simulink model "ids_android_app"  (R2024a)
settings: Solver=FixedStepDiscrete  StartTime=0.0  StopTime=inf  FixedStep=0.1  RelTol=1e-3
libraries: androiduilib x9, androidsensorlib x4, androidcommunicationlib x2, androidaudiovideolib x1
settings Model: Creator=prana  LastModifiedBy=prana
settings OptimizationCC: EnhancedBackFolding=on  PassReuseOutputArgsAs=Individual arguments  ZeroExternalMemoryAtStartup=off  ZeroInternalMemoryAtStartup=off  MaxStackSize=64  OptimizeBlockOrder=speed  DifferentSizesBufferReuse=on  OptimizationCustomize=off  EfficientTunableParamExpr=on
settings DebuggingCC: ParameterTunabilityLossMsg=error
settings HardwareCC: ProdBitPerPointer=32  ProdBitPerSizeT=32  ProdBitPerPtrDiffT=32  ProdLargestAtomicInteger=Long  ProdLargestAtomicFloat=Double  ProdWordSize=32  ProdHWDeviceType=ARM Compatible->ARM Cortex  UseEmbeddedCoderFeatures=off  UseSimulinkCoderFeatures=off
settings SFSimCC: MATLABDynamicMemAlloc=off
settings RTWCC: Description=Embedded Coder  SystemTargetFile=ert.tlc  HardwareBoard=Android Device  TLCOptions="-aInlineSetEventsForThisBaseRateFcn=TLC_FALSE -aSuppressMultiTaskScheduler=TLC_FALSE  -aRateBasedStepFcn=0"  TemplateMakefile=ert_default_tmf  RTWVerbose=off  Toolchain=Android SDK/NDK Tools
settings CodeAppCC: ForceParamTrailComments=on  IgnoreCustomStorageClasses=off  OperatorAnnotations=on  SimulinkDataObjDesc=on  SFDataObjDesc=on  InsertBlockDesc=on
settings ERTTargetCC: SupportNonInlinedSFcns=on

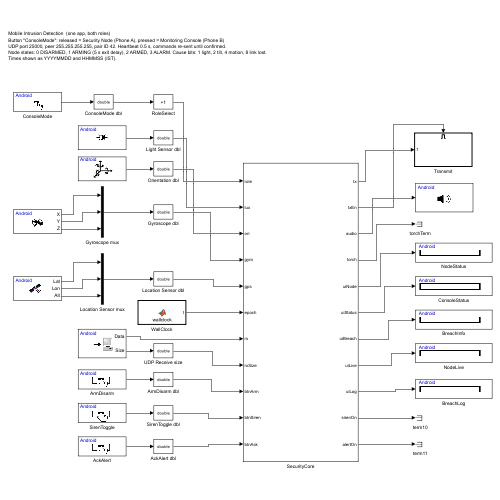
[thumbnail: Simulink's stored preview of the top-level diagram]
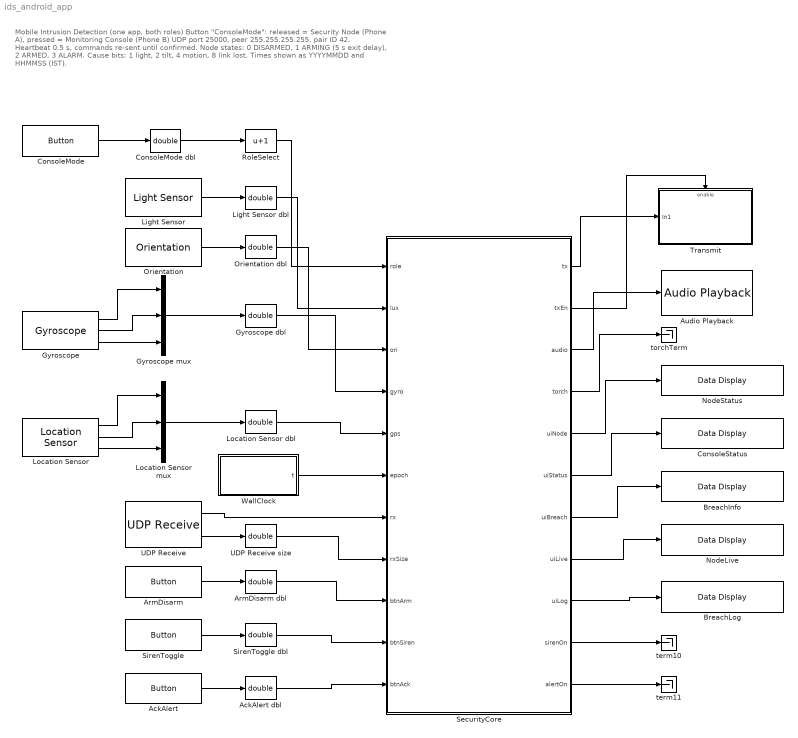
== system ids_android_app ==
  note: Mobile Intrusion Detection  (one app, both roles)
      | Button "ConsoleMode": released = Security Node (Phone A), pressed = Monitoring Console (Phone B)
      | UDP port 25000, peer 255.255.255.255, pair ID 42. Heartbeat 0.5 s, commands re-sent until confirmed.
      | Node states: 0 DISARMED, 1 ARMING (5 s exit delay), 2 ARMED, 3 ALARM. Cause bits: 1 light, 2 tilt, 4 motion, 8 link lost.
      | Times shown as YYYYMMDD and HHMMSS (IST).
  AckAlert : androiduilib/Button  ButtonState=Not pressed  ButtonId=ids_android_app/AckAlert  State=off  SampleTime=0.1  BlockPlatform=Android
  AckAlert dbl : DataTypeConversion  OutDataTypeStr=double  SaturateOnIntegerOverflow=off  RndMeth=Floor
  ArmDisarm : androiduilib/Button  ButtonState=Not pressed  ButtonId=ids_android_app/ArmDisarm  State=off  SampleTime=0.1  BlockPlatform=Android
  ArmDisarm dbl : DataTypeConversion  OutDataTypeStr=double  SaturateOnIntegerOverflow=off  RndMeth=Floor
  Audio Playback : androidaudiovideolib/Audio Playback  SampleFreq=44100  AudioSamplingFreq=44100  SampleTime=0.1  DeviceStr=0  QueueDuration=0  BlockPlatform=Android
  BreachInfo : androiduilib/Data Display  DataDisplayId=ids_android_app/BreachInfo  Format=Float  Precision=6  SimulateUsing=Code generation  blockPlatform=Android
  BreachLog : androiduilib/Data Display  DataDisplayId=ids_android_app/BreachLog  Format=Float  Precision=6  SimulateUsing=Code generation  blockPlatform=Android
  ConsoleMode : androiduilib/Button  ButtonState=Not pressed  ButtonId=ids_android_app/ConsoleMode  State=off  SampleTime=0.1  BlockPlatform=Android
  ConsoleMode dbl : DataTypeConversion  OutDataTypeStr=double  SaturateOnIntegerOverflow=off  RndMeth=Floor
  ConsoleStatus : androiduilib/Data Display  DataDisplayId=ids_android_app/ConsoleStatus  Format=Float  Precision=6  SimulateUsing=Code generation  blockPlatform=Android
  Gyroscope : androidsensorlib/Gyroscope  OutputVector=off  SampleTime=0.1  BlockPlatform=Android
  Gyroscope dbl : DataTypeConversion  OutDataTypeStr=double  SaturateOnIntegerOverflow=off  RndMeth=Floor
  Gyroscope mux : Mux  Inputs=3
  Light Sensor : androidsensorlib/Light Sensor  SampleTime=0.1  BlockPlatform=Android
  Light Sensor dbl : DataTypeConversion  OutDataTypeStr=double  SaturateOnIntegerOverflow=off  RndMeth=Floor
  Location Sensor : androidsensorlib/Location Sensor  OutputVector=off  SampleTime=0.1  BlockPlatform=Android
  Location Sensor dbl : DataTypeConversion  OutDataTypeStr=double  SaturateOnIntegerOverflow=off  RndMeth=Floor
  Location Sensor mux : Mux  Inputs=3
  NodeLive : androiduilib/Data Display  DataDisplayId=ids_android_app/NodeLive  Format=Float  Precision=6  SimulateUsing=Code generation  blockPlatform=Android
  NodeStatus : androiduilib/Data Display  DataDisplayId=ids_android_app/NodeStatus  Format=Float  Precision=6  SimulateUsing=Code generation  blockPlatform=Android
  Orientation : androidsensorlib/Orientation  SampleTime=0.1
  Orientation dbl : DataTypeConversion  OutDataTypeStr=double  SaturateOnIntegerOverflow=off  RndMeth=Floor
  RoleSelect : Bias  Bias=1  SaturateOnIntegerOverflow=off
  SecurityCore : Subsystem
  SirenToggle : androiduilib/Button  ButtonState=Not pressed  ButtonId=ids_android_app/SirenToggle  State=off  SampleTime=0.1  BlockPlatform=Android
  SirenToggle dbl : DataTypeConversion  OutDataTypeStr=double  SaturateOnIntegerOverflow=off  RndMeth=Floor
  Transmit : Subsystem  TreatAsAtomicUnit=on
  UDP Receive : androidcommunicationlib/UDP Receive  localURL='0.0.0.0'  localPort=25000  remoteURL='0.0.0.0'  remotePort=-1  recvBufferSize=1024  signalDatatype=double  dims=16  isVarSize=off  showBlockingTime=off  blockingTime=0  sampletime=0.1  blockPlatform=Android
  UDP Receive size : DataTypeConversion  OutDataTypeStr=double  SaturateOnIntegerOverflow=off  RndMeth=Floor
  WallClock : MATLAB Function  TreatAsAtomicUnit=on
  term10 : Terminator
  term11 : Terminator
  torchTerm : Terminator
  wires:
  ConsoleMode/1 -> ConsoleMode dbl/1
  SecurityCore/5(uiNode) -> NodeStatus/1
  Gyroscope/2 -> Gyroscope mux/2
  Gyroscope/1 -> Gyroscope mux/1
  Gyroscope/3 -> Gyroscope mux/3
  ConsoleMode dbl/1 -> RoleSelect/1
  Gyroscope dbl/1 -> SecurityCore/4(gyro)
  Gyroscope mux/1 -> Gyroscope dbl/1
  Location Sensor/3 -> Location Sensor mux/3
  Location Sensor/2 -> Location Sensor mux/2
  Location Sensor/1 -> Location Sensor mux/1
  Light Sensor/1 -> Light Sensor dbl/1
  SecurityCore/7(uiBreach) -> BreachInfo/1
  Orientation/1 -> Orientation dbl/1
  ArmDisarm dbl/1 -> SecurityCore/9(btnArm)
  Location Sensor mux/1 -> Location Sensor dbl/1
  UDP Receive/1 -> SecurityCore/7(rx)
  UDP Receive/2 -> UDP Receive size/1
  ArmDisarm/1 -> ArmDisarm dbl/1
  SirenToggle/1 -> SirenToggle dbl/1
  SirenToggle dbl/1 -> SecurityCore/10(btnSiren)
  AckAlert/1 -> AckAlert dbl/1
  RoleSelect/1 -> SecurityCore/1(role)
  SecurityCore/8(uiLive) -> NodeLive/1
  SecurityCore/4(torch) -> torchTerm/1
  Light Sensor dbl/1 -> SecurityCore/2(lux)
  Orientation dbl/1 -> SecurityCore/3(ori)
  Location Sensor dbl/1 -> SecurityCore/5(gps)
  WallClock/1(t) -> SecurityCore/6(epoch)
  UDP Receive size/1 -> SecurityCore/8(rxSize)
  AckAlert dbl/1 -> SecurityCore/11(btnAck)
  SecurityCore/1(tx) -> Transmit/1(In1)
  SecurityCore/2(txEn) -> Transmit/Enable
  SecurityCore/3(audio) -> Audio Playback/1
  SecurityCore/6(uiStatus) -> ConsoleStatus/1
  SecurityCore/9(uiLog) -> BreachLog/1
  SecurityCore/10(sirenOn) -> term10/1
  SecurityCore/11(alertOn) -> term11/1

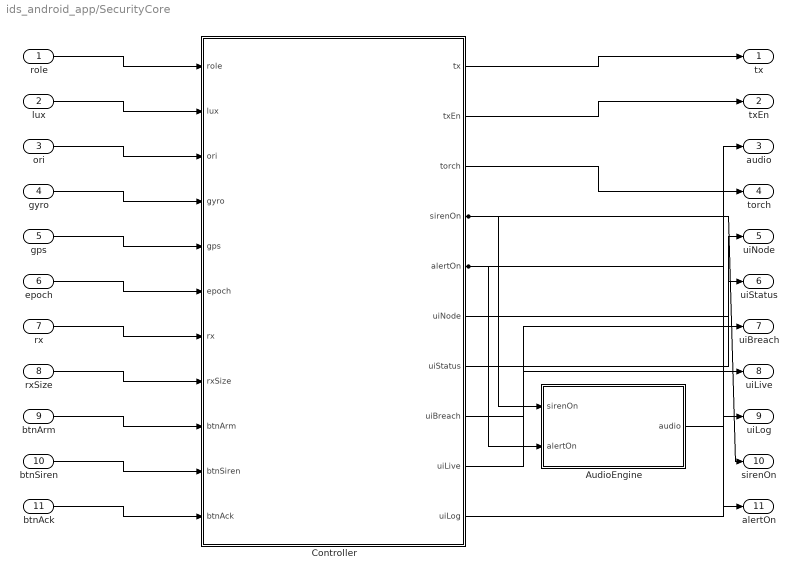
== system ids_android_app/SecurityCore ==
  role : Inport
  lux : Inport  Port=2
  ori : Inport  Port=3
  gyro : Inport  Port=4
  gps : Inport  Port=5
  epoch : Inport  Port=6
  rx : Inport  Port=7
  rxSize : Inport  Port=8
  btnArm : Inport  Port=9
  btnSiren : Inport  Port=10
  btnAck : Inport  Port=11
  AudioEngine : MATLAB Function  TreatAsAtomicUnit=on
  Controller : MATLAB Function  TreatAsAtomicUnit=on
  tx : Outport
  txEn : Outport  Port=2
  audio : Outport  Port=3
  torch : Outport  Port=4
  uiNode : Outport  Port=5
  uiStatus : Outport  Port=6
  uiBreach : Outport  Port=7
  uiLive : Outport  Port=8
  uiLog : Outport  Port=9
  sirenOn : Outport  Port=10
  alertOn : Outport  Port=11
  wires:
  role/1 -> Controller/1(role)
  lux/1 -> Controller/2(lux)
  ori/1 -> Controller/3(ori)
  gyro/1 -> Controller/4(gyro)
  gps/1 -> Controller/5(gps)
  epoch/1 -> Controller/6(epoch)
  rx/1 -> Controller/7(rx)
  rxSize/1 -> Controller/8(rxSize)
  btnArm/1 -> Controller/9(btnArm)
  btnSiren/1 -> Controller/10(btnSiren)
  btnAck/1 -> Controller/11(btnAck)
  Controller/1(tx) -> tx/1
  Controller/2(txEn) -> txEn/1
  Controller/3(torch) -> torch/1
  Controller/4(sirenOn) -> AudioEngine/1(sirenOn), sirenOn/1
  Controller/5(alertOn) -> AudioEngine/2(alertOn), alertOn/1
  Controller/6(uiNode) -> uiNode/1
  Controller/7(uiStatus) -> uiStatus/1
  Controller/8(uiBreach) -> uiBreach/1
  Controller/9(uiLive) -> uiLive/1
  Controller/10(uiLog) -> uiLog/1
  AudioEngine/1(audio) -> audio/1

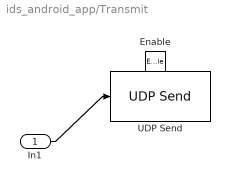
== system ids_android_app/Transmit ==
  In1 : Inport
  Enable : EnablePort
  UDP Send : androidcommunicationlib/UDP Send  remoteURL='255.255.255.255'  remotePort=25000  localURL='0.0.0.0'  localPortSource=Automatically determine  localPort=-1  sampletime=-1  blockPlatform=Android  separateLengthPort=0
  wires:
  In1/1 -> UDP Send/1

== matlab function ids_android_app/SecurityCore/AudioEngine ==
  data: sirenOn input; audio output; alertOn input
function audio = audio_engine(sirenOn, alertOn)
%#codegen
P = coder.const(ids_params());
persistent A                      % audio state kept between steps
if isempty(A)
    A = audio_init();
end
% coder.load reads alert_message.mat while the code is being generated, so
% the recorded message becomes a constant array inside the app.
S = coder.load('alert_message.mat', 'msg');
[A, audio] = audio_step(A, sirenOn, alertOn, S.msg, P);
end

== matlab function ids_android_app/SecurityCore/Controller ==
  data: role input; tx output; lux input; ori input; gyro input; gps input; epoch input; rx input; rxSize input; btnArm input; btnSiren input; btnAck input; txEn output; torch output; sirenOn output; alertOn output; uiNode output; uiStatus output; uiBreach output; uiLive output; uiLog output
function [tx, txEn, torch, sirenOn, alertOn, uiNode, uiStatus, uiBreach, uiLive, uiLog] = controller(role, lux, ori, gyro, gps, epoch, rx, rxSize, btnArm, btnSiren, btnAck)
%#codegen
% Runs the Security Node and the Monitoring Console logic. Only the role
% selected by "role" is active, the other one is held in reset.
% Load the constants once at compile time so they become C literals.
P = coder.const(ids_params());
% "persistent" = a C static variable. Values survive between calls, which
% is how the block remembers its state from one 0.1 s step to the next.
persistent N C
if isempty(N)                     % true only on the very first call
    N = node_init();
    C = console_init(P.logLen);
end
% role comes from the Button: 1 = node, 2 = console. Comparing with 1.5 is
% robust to float or integer typing of the signal.
isNode = double(role(1)) < 1.5;
% Convert Simulink signals to plain doubles for the step functions.
rxd = double(rx(:));
rxs = double(rxSize(1));
t   = double(epoch(1));
% Both state machines run every step. The inactive one gets active = false
% and just resets itself. The transpose (apostrophe) makes row vectors.
[N, txN, enN, torchD, uiNode] = node_step(N, isNode, double(lux(1)), double(ori(:)'), double(gyro(:)'), double(gps(:)'), t, rxd, rxs, P);
[C, txC, enC, uiStatus, uiBreach, uiLive, uiLog] = console_step(C, ~isNode, double(btnArm(1)), double(btnSiren(1)), double(btnAck(1)), t, rxd, rxs, P);
% Pick the packet of the active role.
if isNode
    tx = txN;
    txEn = enN;
else
    tx = txC;
    txEn = enC;
end
% Outputs for the rest of the diagram. The Android ToApp block needs an int32.
torch   = int32(torchD);
sirenOn = double(isNode && N.siren > 0);
alertOn = double(~isNode && C.alert > 0);
end

== matlab function ids_android_app/WallClock ==
  settings: updateMethod=DISCRETE  sampleTime=0.1
  data: t output
function t = wallclock()
% Unix time from the phone clock (time(NULL) in the generated C)
t = wall_clock();
